simulink model "apf_vps_H3"  (R2025a)
settings: Solver=FixedStepDiscrete  StartTime=0.0  StopTime=T_end  FixedStep=V.H  RelTol=1e-3
PostLoadFcn:
  | addpath(fileparts(get_param('apf_vps_H3','FileName'))); if ~exist('P','var'), run(fullfile(fileparts(get_param('apf_vps_H3','FileName')),'apf_params.m')); end; if ~exist('V','var'), V = vps_params_H3(true); end
InitFcn:
  | addpath(fileparts(get_param('apf_vps_H3','FileName'))); if ~exist('P','var'), run(fullfile(fileparts(get_param('apf_vps_H3','FileName')),'apf_params.m')); end; if ~exist('V','var'), V = vps_params_H3(true); end
values from neighbouring files (symbols this model uses):
  dtc = Td / (Ts / 2) / 2    [apf_params.m]    (also in vps_vectors_H3.m = 0.02)
  T_log = 10e-6    (= 1e-05)    [apf_params.m]
  t_run = 0.01    [apf_params.m]
  t_step = 0.7    [apf_params.m]
  Ts = P.Ts    [apf_params.m]    (also in sensor_params_H2.m = 0.0001)
  V = vps_params_H3(false) -> real numbers.\n'      'Waveforms scope: grid voltage, grid current, load current, inverter current, DC link. Run matlab/vps_check_H3.m for the comparison.'])    [build_apf_vps_H3.m]    (also in vps_check_H3.m = vps_params_H3(fx); vps_vectors_H3.m = vps_params_H3(true); vps_walkthrough_H3.m = vps_params_H3(true))
libraries: simulink x1
settings Model: Creator=HeKe  LastModifiedBy=HeKe

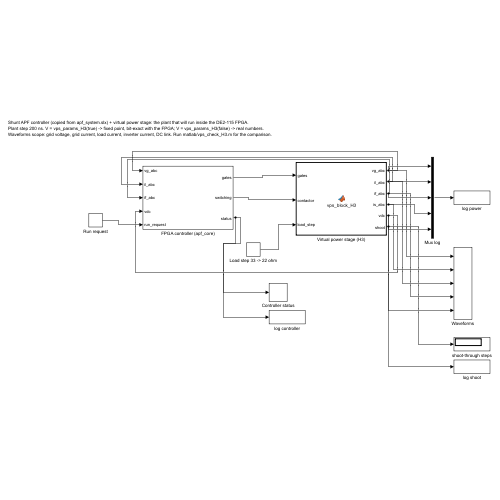
[thumbnail: Simulink's stored preview of the top-level diagram]
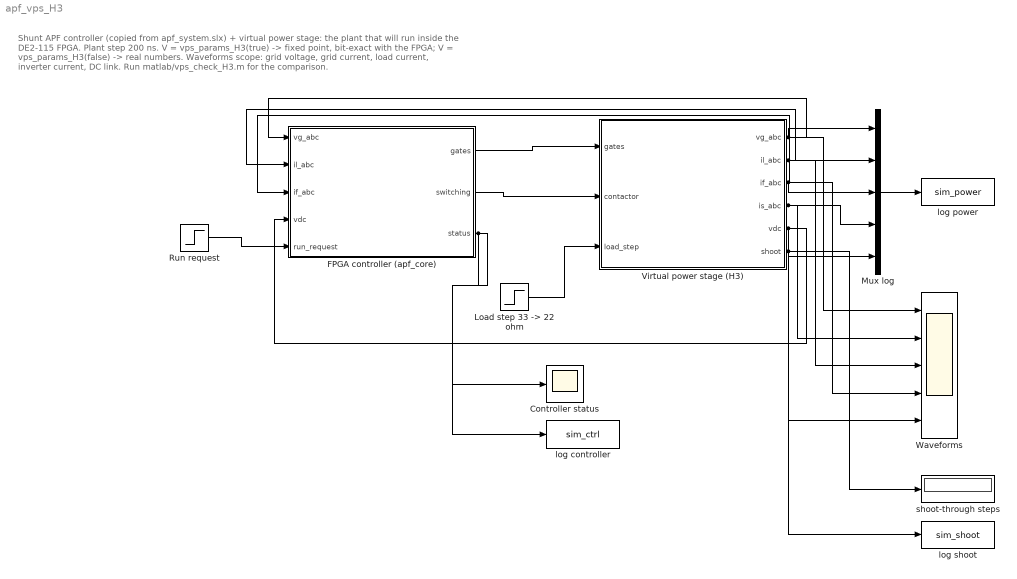
== system apf_vps_H3 ==
  note: Shunt APF controller (copied from apf_system.slx) + virtual power stage: the plant that will run inside the DE2-115 FPGA.
      | Plant step 200 ns. V = vps_params_H3(true) -> fixed point, bit-exact with the FPGA; V = vps_params_H3(false) -> real numbers.
      | Waveforms scope: grid voltage, grid current, load current, inverter current, DC link. Run matlab/vps_check_H3.m for the comparison.
  Controller status : Scope
  FPGA controller (apf_core) : Subsystem
  "Load step 33 -> 22 ohm" : Step  Time=t_step  SampleTime=Ts
  Mux log : Mux  Inputs=[3 3 3 3 1]
  Run request : Step  Time=t_run  SampleTime=Ts
  Virtual power stage (H3) : MATLAB Function  TreatAsAtomicUnit=on  SystemSampleTime=V.H
  Waveforms : Scope  NumInputPorts=5
  log controller : ToWorkspace  VariableName=sim_ctrl  SaveFormat=Structure With Time  SampleTime=Ts
  log power : ToWorkspace  VariableName=sim_power  SaveFormat=Structure With Time  SampleTime=T_log
  log shoot : ToWorkspace  VariableName=sim_shoot  SampleTime=Ts
  shoot-through steps : Display
  wires:
  FPGA controller (apf_core)/1(gates) -> Virtual power stage (H3)/1(gates)
  FPGA controller (apf_core)/2(switching) -> Virtual power stage (H3)/2(contactor)
  "Load step 33 -> 22 ohm"/1 -> Virtual power stage (H3)/3(load_step)
  Virtual power stage (H3)/1(vg_abc) -> FPGA controller (apf_core)/1(vg_abc), Mux log/1, Waveforms/1
  Virtual power stage (H3)/2(il_abc) -> FPGA controller (apf_core)/2(il_abc), Mux log/2, Waveforms/3
  Virtual power stage (H3)/3(if_abc) -> FPGA controller (apf_core)/3(if_abc), Mux log/3, Waveforms/4
  Virtual power stage (H3)/5(vdc) -> FPGA controller (apf_core)/4(vdc), Mux log/5, Waveforms/5
  Run request/1 -> FPGA controller (apf_core)/5(run_request)
  Virtual power stage (H3)/4(is_abc) -> Mux log/4, Waveforms/2
  Mux log/1 -> log power/1
  Virtual power stage (H3)/6(shoot) -> shoot-through steps/1, log shoot/1
  FPGA controller (apf_core)/3(status) -> Controller status/1, log controller/1

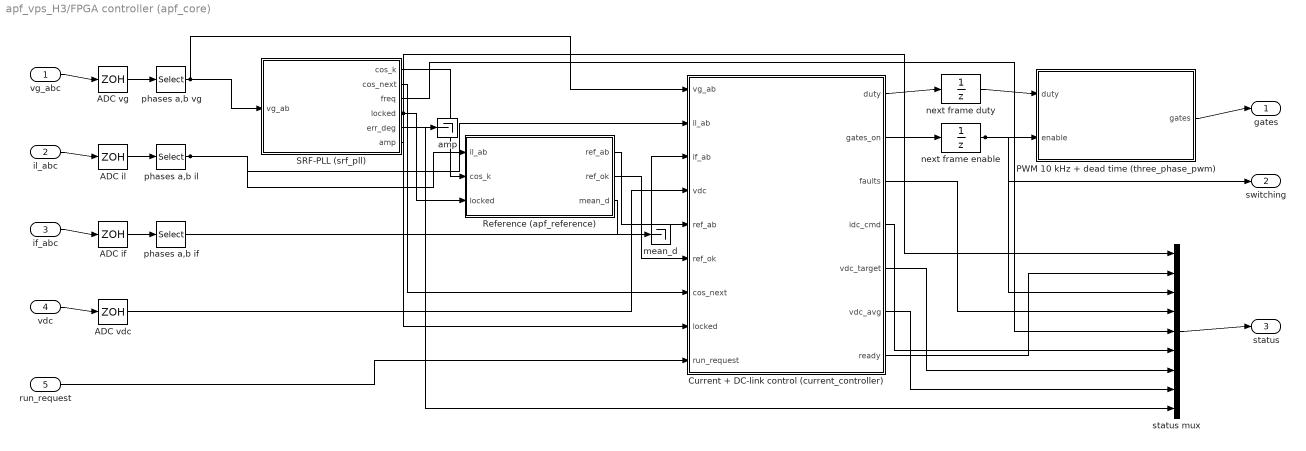
== system apf_vps_H3/FPGA controller (apf_core) ==
  vg_abc : Inport
  il_abc : Inport  Port=2
  if_abc : Inport  Port=3
  vdc : Inport  Port=4
  run_request : Inport  Port=5
  ADC if : ZeroOrderHold  SampleTime=Ts
  ADC il : ZeroOrderHold  SampleTime=Ts
  ADC vdc : ZeroOrderHold  SampleTime=Ts
  ADC vg : ZeroOrderHold  SampleTime=Ts
  Current + DC-link control (current_controller) : MATLAB Function  TreatAsAtomicUnit=on
  PWM 10 kHz + dead time (three_phase_pwm) : Subsystem
  Reference (apf_reference) : MATLAB Function  TreatAsAtomicUnit=on
  SRF-PLL (srf_pll) : MATLAB Function  TreatAsAtomicUnit=on
  amp : Terminator
  mean_d : Terminator
  next frame duty : UnitDelay  SampleTime=Ts  HasFrameUpgradeWarning=on
  next frame enable : UnitDelay  SampleTime=Ts  HasFrameUpgradeWarning=on
  phases a,b if : Selector  InputPortWidth=3  IndexOptions=Index vector (dialog)  Indices=[1 2]  OutputSizes=1
  phases a,b il : Selector  InputPortWidth=3  IndexOptions=Index vector (dialog)  Indices=[1 2]  OutputSizes=1
  phases a,b vg : Selector  InputPortWidth=3  IndexOptions=Index vector (dialog)  Indices=[1 2]  OutputSizes=1
  status mux : Mux  Inputs=9
  gates : Outport
  switching : Outport  Port=2
  status : Outport  Port=3
  wires:
  Reference (apf_reference)/3(mean_d) -> mean_d/1
  SRF-PLL (srf_pll)/6(amp) -> amp/1
  status mux/1 -> status/1
  SRF-PLL (srf_pll)/5(err_deg) -> status mux/9
  Current + DC-link control (current_controller)/6(vdc_avg) -> status mux/8
  Current + DC-link control (current_controller)/5(vdc_target) -> status mux/7
  Current + DC-link control (current_controller)/4(idc_cmd) -> status mux/6
  SRF-PLL (srf_pll)/3(freq) -> status mux/5
  Current + DC-link control (current_controller)/3(faults) -> status mux/4
  Current + DC-link control (current_controller)/7(ready) -> status mux/2
  PWM 10 kHz + dead time (three_phase_pwm)/1(gates) -> gates/1
  next frame enable/1 -> status mux/3, switching/1, PWM 10 kHz + dead time (three_phase_pwm)/2(enable)
  next frame duty/1 -> PWM 10 kHz + dead time (three_phase_pwm)/1(duty)
  Current + DC-link control (current_controller)/2(gates_on) -> next frame enable/1
  Current + DC-link control (current_controller)/1(duty) -> next frame duty/1
  run_request/1 -> Current + DC-link control (current_controller)/9(run_request)
  SRF-PLL (srf_pll)/2(cos_next) -> Current + DC-link control (current_controller)/7(cos_next)
  Reference (apf_reference)/2(ref_ok) -> Current + DC-link control (current_controller)/6(ref_ok)
  Reference (apf_reference)/1(ref_ab) -> Current + DC-link control (current_controller)/5(ref_ab)
  ADC vdc/1 -> Current + DC-link control (current_controller)/4(vdc)
  phases a,b if/1 -> Current + DC-link control (current_controller)/3(if_ab)
  SRF-PLL (srf_pll)/4(locked) -> status mux/1, Current + DC-link control (current_controller)/8(locked), Reference (apf_reference)/3(locked)
  SRF-PLL (srf_pll)/1(cos_k) -> Reference (apf_reference)/2(cos_k)
  phases a,b il/1 -> Current + DC-link control (current_controller)/2(il_ab), Reference (apf_reference)/1(il_ab)
  phases a,b vg/1 -> Current + DC-link control (current_controller)/1(vg_ab), SRF-PLL (srf_pll)/1(vg_ab)
  vdc/1 -> ADC vdc/1
  ADC if/1 -> phases a,b if/1
  if_abc/1 -> ADC if/1
  ADC il/1 -> phases a,b il/1
  il_abc/1 -> ADC il/1
  ADC vg/1 -> phases a,b vg/1
  vg_abc/1 -> ADC vg/1

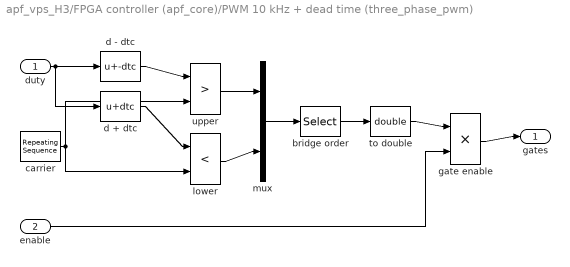
== system apf_vps_H3/FPGA controller (apf_core)/PWM 10 kHz + dead time (three_phase_pwm) ==
  duty : Inport
  enable : Inport  Port=2
  bridge order : Selector  InputPortWidth=6  IndexOptions=Index vector (dialog)  Indices=[1 4 2 5 3 6]  OutputSizes=1
  carrier : simulink/Sources/Repeating Sequence  rep_seq_t=[0 Ts/2 Ts]  rep_seq_y=[0 1 0]
  d + dtc : Bias  Bias=dtc  SaturateOnIntegerOverflow=off
  d - dtc : Bias  Bias=-dtc  SaturateOnIntegerOverflow=off
  gate enable : Product
  lower : RelationalOperator  Operator=<  OutDataTypeStr=boolean  RndMeth=Simplest  InputSameDT=off
  mux : Mux  Inputs=2
  to double : DataTypeConversion  OutDataTypeStr=double  SaturateOnIntegerOverflow=off  RndMeth=Floor
  upper : RelationalOperator  Operator=>  OutDataTypeStr=boolean  RndMeth=Simplest  InputSameDT=off
  gates : Outport
  wires:
  gate enable/1 -> gates/1
  enable/1 -> gate enable/2
  to double/1 -> gate enable/1
  bridge order/1 -> to double/1
  mux/1 -> bridge order/1
  lower/1 -> mux/2
  upper/1 -> mux/1
  d + dtc/1 -> lower/1
  carrier/1 -> lower/2, upper/2
  d - dtc/1 -> upper/1
  duty/1 -> d + dtc/1, d - dtc/1

== matlab function apf_vps_H3/FPGA controller (apf_core)/Reference (apf_reference) ==
  data: il_ab input; ref_ab output; cos_k input; locked input; ref_ok output; mean_d output; P parameter
function [ref_ab, ref_ok, mean_d] = apf_reference_block(il_ab, cos_k, locked, P)
% Compensation reference, floating-point equivalent of rtl/apf_reference.sv.
%   d      = 2/3 * sum(i_load_p * cos_p)       (active load current, this sample)
%   mean_d = average of d over one grid cycle   (N samples)
%   ref_p  = i_load_p - mean_d * cos_p          (harmonics + reactive current)
% The history is discarded whenever the PLL is not locked.
persistent hist idx cnt total
NMAX = 400;                       % buffer size; P.N must not exceed it
if isempty(hist)
    hist = zeros(1, NMAX); idx = 1; cnt = 0; total = 0;
end
ref_ab = [0, 0];
ref_ok = 0;
mean_d = 0;
if locked < 0.5
    hist(:) = 0; idx = 1; cnt = 0; total = 0;
    return;
end
N = P.N;
il = [il_ab(1), il_ab(2), -(il_ab(1) + il_ab(2))];
d = 2/3 * sum(il .* cos_k);

% Rolling sum over the last N samples.
if cnt == N
    total = total - hist(idx);
end
total = total + d;
hist(idx) = d;
idx = idx + 1;
if idx > N, idx = 1; end
cnt = min(cnt + 1, N);

if cnt == N
    mean_d = total / N;
    ref_ab = il(1:2) - mean_d * cos_k(1:2);
    ref_ok = 1;
end

== matlab function apf_vps_H3/FPGA controller (apf_core)/SRF-PLL (srf_pll) ==
  data: vg_ab input; cos_k output; cos_next output; freq output; locked output; err_deg output; amp output; P parameter
function [cos_k, cos_next, freq, locked, err_deg, amp] = srf_pll_block(vg_ab, P)
% Three-phase SRF-PLL, floating-point equivalent of rtl/srf_pll.sv
% (bit-exact integer model: model/pll_model.py). Runs once per control frame.
%   cos_k    cosines of the angle predicted for this sample (used by the reference)
%   cos_next cosines for the next sample (used by the current controller)
persistent theta integ is_locked lock_cnt unlock_cnt
if isempty(theta)
    theta = 0; integ = 0; is_locked = false; lock_cnt = 0; unlock_cnt = 0;
end
sh = [0, -2*pi/3, 2*pi/3];
vabc = [vg_ab(1), vg_ab(2), -(vg_ab(1) + vg_ab(2))];

% 1. Park transform with the predicted angle.
c = cos(theta + sh);
s = sin(theta + sh);
vd = 2/3 * sum(vabc .* c);
vq = -2/3 * sum(vabc .* s);

% 2. Normalise q by the magnitude: error = sin(phase error).
amp = sqrt(vd^2 + vq^2);
low_amp = amp < P.pll_vmin;
e = 0;
if ~low_amp
    e = vq / amp;
end

% 3. PI loop with frequency clamp and anti-windup.
wn = 2*pi*P.pll_bw;
kp = 2*P.pll_zeta*wn;
ki = wn^2;
imax = 2*pi*(P.pll_fmax - P.f);
integ = min(max(integ + ki*e*P.Ts, -imax), imax);
w = min(max(2*pi*P.f + kp*e + integ, 2*pi*P.pll_fmin), 2*pi*P.pll_fmax);

% 4. Advance the angle for the next sample.
theta = mod(theta + w*P.Ts, 2*pi);

% 5. Lock detection.
good = ~low_amp && abs(e) <= sin(P.lock_deg*pi/180);
bad  = low_amp || abs(e) > sin(P.unlock_deg*pi/180);
if ~is_locked
    if good, lock_cnt = lock_cnt + 1; else, lock_cnt = 0; end
    if lock_cnt >= P.lock_n
        is_locked = true; unlock_cnt = 0;
    end
else
    if bad, unlock_cnt = unlock_cnt + 1; else, unlock_cnt = 0; end
    if unlock_cnt >= P.unlock_n
        is_locked = false; lock_cnt = 0;
    end
end

cos_k = c;
cos_next = cos(theta + sh);
freq = w / (2*pi);
locked = double(is_locked);
err_deg = asin(e) * 180/pi;

== matlab function apf_vps_H3/FPGA controller (apf_core)/Current + DC-link control (current_controller) ==
  data: vg_ab input; duty output; il_ab input; if_ab input; vdc input; ref_ab input; ref_ok input; cos_next input; locked input; run_request input; gates_on output; faults output; idc_cmd output; vdc_target output; vdc_avg output; ready output; P parameter
function [duty, gates_on, faults, idc_cmd, vdc_target, vdc_avg, ready] = apf_control_block( ...
    vg_ab, il_ab, if_ab, vdc, ref_ab, ref_ok, cos_next, locked, run_request, P)
% Predictive (deadbeat) current control, DC-link loop, protection and start-up
% sequencing: floating-point equivalent of rtl/current_controller.sv and the
% sequencing in rtl/apf_core.sv. Runs once per control frame k.
%   duty     upper-switch on fraction per phase, applied over [k+1, k+2]
%   gates_on inverter switching (and contactor) enable for the same interval
%   faults   latched [measurement, over_current, over_voltage, pll_lost]
persistent raw vg_prev hist wr fill vdc_sum vdc_cnt avg vdc_avg_ok integ idc vtgt fresh run_ctrl fault_q
NMAX = 400;
if isempty(raw)
    raw = [0.5, 0.5, 0.5]; vg_prev = [0, 0];
    hist = zeros(2, NMAX); wr = 1; fill = 0;
    vdc_sum = 0; vdc_cnt = 0; avg = 0; vdc_avg_ok = false;
    integ = 0; idc = 0; vtgt = 0;
    fresh = true; run_ctrl = false; fault_q = false(1, 4);
end
N = P.N; Ts = P.Ts; L = P.Lf;
vg3 = [vg_ab(1), vg_ab(2), -(vg_ab(1) + vg_ab(2))];
il3 = [il_ab(1), il_ab(2), -(il_ab(1) + il_ab(2))];
if3 = [if_ab(1), if_ab(2), -(if_ab(1) + if_ab(2))];

% ---- protection and sequencing (apf_core) ----
fault_now = [any(abs(vg3(1:2)) > P.v_range) || any(abs(il3(1:2)) > P.i_range) || ...
                 any(abs(if3(1:2)) > P.i_range), ...
             any(abs(if3) > P.i_trip), ...
             vdc > P.vdc_trip, ...
             run_ctrl && locked < 0.5];
% The controller sees the run decision registered in an earlier frame.
run_q = run_ctrl && fill == N && ref_ok > 0.5 && vdc_avg_ok;
if run_request < 0.5
    run_ctrl = false;                     % dropping the request clears faults
    fault_q(:) = false;
elseif any(fault_q) || any(fault_now)
    fault_q = fault_q | fault_now;        % latch, stop switching
    run_ctrl = false;
elseif ~run_ctrl && fill == N && vdc_avg_ok && locked > 0.5
    run_ctrl = true;
end
run_q = run_q && run_ctrl;

% ---- 1. predict the filter current at k+1 ----
dv = vg_ab(:)' - vg_prev;
u_prev = vdc * (raw(1:2) - mean(raw));    % differential voltage applied over [k, k+1]
e1 = u_prev - vg_ab(:)' - dv/2;
if fresh                                   % inverter was not switching over [k, k+1]
    i_pred = if_ab(:)';
else
    i_pred = if_ab(:)' + Ts/L * e1;
end
i_pred3 = [i_pred, -(i_pred(1) + i_pred(2))];

% ---- 2. reference for k+2: one grid cycle earlier, minus the DC-link term ----
rd = wr + P.pred_lead;
if rd > N, rd = rd - N; end
rp = hist(:, rd)' - idc * cos_next(1:2);

% ---- 3. deadbeat voltage with grid feed-forward ----
u = vg_ab(:)' + 1.5*dv + P.G * L/Ts * (rp - i_pred);
u3 = [u, -(u(1) + u(2))];

% ---- 4. min/max common-mode injection, divide by Vdc, dead-time compensation ----
off = -(max(u3) + min(u3)) / 2;
vdc_div = max(vdc, P.vdc_min_div);
raw_n = min(max(0.5 + (u3 + off) / vdc_div, 0), 1);
vg_prev = vg_ab(:)';
if run_q
    raw = raw_n;
    duty = min(max(raw_n + P.Td/Ts * (2*(i_pred3 > 0) - 1), 0), 1);
    fresh = false;
else
    raw = [0.5, 0.5, 0.5];
    duty = [0.5, 0.5, 0.5];
    fresh = true;
end
gates_on = double(run_q);

% ---- store this frame's reference; drop the history if it is broken ----
if ref_ok > 0.5
    hist(:, wr) = ref_ab(:);
    wr = wr + 1;
    if wr > N, wr = 1; end
    fill = min(fill + 1, N);
else
    wr = 1; fill = 0;
end

% ---- DC-link PI, once per grid cycle on the cycle average ----
vdc_sum = vdc_sum + vdc;
vdc_cnt = vdc_cnt + 1;
if vdc_cnt == N
    avg = vdc_sum / N;
    vdc_sum = 0; vdc_cnt = 0; vdc_avg_ok = true;
    if ~run_q
        vtgt = avg; integ = 0; idc = 0;
    else
        vtgt = min(vtgt + P.vdc_ramp * N * Ts, P.vdc_ref);
        err = vtgt - avg;
        integ = min(max(integ + P.ki_dc * err * N * Ts, -P.idc_max), P.idc_max);
        idc = min(max(P.kp_dc * err + integ, -P.idc_max), P.idc_max);
    end
end

faults = double(fault_q);
idc_cmd = idc;
vdc_target = vtgt;
vdc_avg = avg;
ready = double(fill == N && vdc_avg_ok && locked > 0.5);

== matlab function apf_vps_H3/Virtual power stage (H3) ==
  data: gates input; vg_abc output; contactor input; load_step input; il_abc output; if_abc output; is_abc output; vdc output; shoot output; V parameter
function [vg_abc, il_abc, if_abc, is_abc, vdc, shoot] = vps_block_H3(gates, contactor, load_step, V)
% H3: virtual power stage, one plant step (H = 200 ns). Equations and number
% formats are specified in vps_params_H3.m; with V.fx = true every operation is
% integer math with the rounding the FPGA uses, so this is the bit-exact
% reference for the FPGA code. With V.fx = false the same equations run with
% exact constants (the real-number reference).
%   gates      [A hi, A lo, B hi, B lo, C hi, C lo] (Universal Bridge order)
%   contactor  inverter connected (the controller's "switching")
%   load_step  0: R1 (33 ohm), 1: R2 (22 ohm)
%   outputs    grid voltage, load current (grid -> load), inverter current
%              (inverter -> grid), grid current (load - inverter), V and A;
%              shoot = number of steps with both switches of a leg on
persistent th vdcq ifq ilq idq nshoot
if isempty(th)
    th = 0; vdcq = V.vdc0_q; ifq = [0 0 0]; ilq = [0 0 0]; idq = 0; nshoot = 0;
end

% ---- grid voltage ----
th = mod(th + V.dth, 2^40);
vg = [0 0 0];
for p = 1:3
    a = mod(th - (p - 1) * V.th120, 2^40);
    vg(p) = rsh(cosine(a, V) * V.Kvm, 16, V.fx);
end

% ---- inverter legs, filter inductors, DC link ----
vdc_v = rsh(vdcq, 12, V.fx);                 % DC link in the voltage format (2^-12 V)
if contactor > 0.5
    vx = [0 0 0];
    for p = 1:3
        hi = gates(2 * p - 1) > 0.5; lo = gates(2 * p) > 0.5;
        if hi && lo, nshoot = nshoot + 1; end
        if hi
            vx(p) = vdc_v;
        elseif lo
            vx(p) = 0;
        elseif ifq(p) > 0                    % dead time: a diode carries the current
            vx(p) = 0;
        else
            vx(p) = vdc_v;
        end
    end
    vn = rsh((vx(1) + vx(2) + vx(3)) * V.K3, 16, V.fx);
    top = 0;
    for p = 1:3
        if vx(p) > 0, top = top + ifq(p); end   % current drawn from the DC link
    end
    for p = 1:2
        dv = vx(p) - vn - vg(p) - rsh(ifq(p) * V.Krf, 28, V.fx);
        ifq(p) = ifq(p) + rsh(dv * V.Kl, 16, V.fx);
    end
    ifq(3) = -(ifq(1) + ifq(2));
    vdcq = vdcq - rsh(top * V.Kc, 24, V.fx) - rsh(vdcq * V.Kleak, 32, V.fx);
else
    for p = 1:6
        if gates(p) > 0.5, nshoot = nshoot + 1; end   % gates must be off
    end
    ifq = [0 0 0];
    vdcq = vdcq - rsh(vdcq * V.Kleak, 32, V.fx);
end

% ---- diode-bridge load ----
imax = 1; imin = 1;
for p = 2:3                                  % first index wins on a tie (deterministic)
    if vg(p) > vg(imax), imax = p; end
    if vg(p) < vg(imin), imin = p; end
end
if load_step > 0.5, R = V.R2; else, R = V.R1; end
idq = idq + rsh((vg(imax) - vg(imin) - rsh(idq * R, 12, V.fx)) * V.Kd, 16, V.fx);
if idq < 0, idq = 0; end
for p = 1:3
    if p == imax
        target = idq;
    elseif p == imin
        target = -idq;
    else
        target = 0;
    end
    ilq(p) = ilq(p) + rsh((target - ilq(p)) * V.Kt, 20, V.fx);
end

vg_abc = vg(:) / 2^12;
il_abc = ilq(:) / 2^24;
if_abc = ifq(:) / 2^24;
is_abc = il_abc - if_abc;
vdc = vdcq / 2^24;
shoot = nshoot;
end


function c = cosine(a, V)
% cos(2*pi*a/2^40) * 2^16: table + linear interpolation (fixed point), exact otherwise
if V.fx
    idx = floor(a / 2^28);                   % top 12 bits
    frac = floor(mod(a, 2^28) / 2^16);       % next 12 bits
    c0 = V.cos_table(idx + 1);
    c1 = V.cos_table(mod(idx + 1, 4096) + 1);
    c = c0 + rsh((c1 - c0) * frac, 12, true);
else
    c = cos(2 * pi * a / 2^40) * 2^16;
end
end


function y = rsh(x, s, fx)
% x / 2^s, rounded half up in fixed point: (x + (1 << (s-1))) >>> s
if fx
    y = floor((x + 2^(s - 1)) / 2^s);
else
    y = x / 2^s;
end
end
